simulink model "ray_motor"  (Simulink 7.7)
settings: Solver=FixedStepDiscrete  SolverMode=SingleTasking  StartTime=0.0  StopTime=inf  FixedStep=0.001  RelTol=1e-3
libraries: dsPICdrivers x9, simulink x1
settings Model: Creator=Ray  LastModifiedBy=l45chen
settings OptimizationCC: OptimizeModelRefInitCode=on  LifeSpan=Inf
settings HardwareCC: ProdBitPerInt=16  ProdBitPerPointer=16  ProdEndianess=LittleEndian  ProdWordSize=16  ProdHWDeviceType=16-bit Generic
settings RTWCC: SystemTargetFile=dspic.tlc  MakeCommand=make_CreateMPLAB  TemplateMakefile=dspic_pic30_gcc.tmf  PostCodeGenCommand=dsPIC_Compile()  Description=Embedded Target for Microchip dsPIC (real-time)  ProcessScript=dspic_make_rtw_hook
settings CodeAppCC: IgnoreCustomStorageClasses=off
settings STFCustomTargetCC: FunctionExecutionProfile=off  IncludeMdlTerminateFcn=off  CombineOutputUpdateFcns=on  ERTCustomFileBanners=on  SupportNonInlinedSFcns=off  SystemTargetFile=dspic.tlc
settings ERTTargetCC: FunctionExecutionProfile=off  MultiwordLength=2048  ParMdlRefBuildCompliant=off  CompOptLevelCompliant=off  IncludeMdlTerminateFcn=off  ERTFirstTimeCompliant=off  SupportContinuousTime=on  ModelStepFunctionPrototypeControlCompliant=off  CPPClassGenCompliant=off  ExtModeMexFile=ext_serial_win32_comm  InlinedParameterPlacement=NonHierarchical  ERTSrcFileBannerTemplate=dsPIC_code_template.cgt  ERTHdrFileBannerTemplate=dsPIC_code_template.cgt  ERTDataSrcFileTemplate=dsPIC_code_template.cgt  ERTDataHdrFileTemplate=dsPIC_code_template.cgt  ERTCustomFileTemplate=dsPIC_main.tlc  ConvertIfToSwitch=off
settings CustomProperty: DataType=string  Value=C:\PROGRA~1\MATLAB\R2011a\bin\win64\gmake

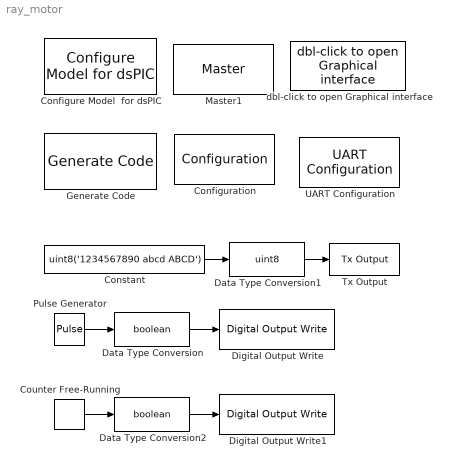
== system ray_motor ==
  Configuration : dsPICdrivers/Configuration  SystemSampleTime=-1  double64=off
  Configure Model  for dsPIC : dsPICdrivers/Simulink Configuration/Configure Model  for dsPIC
  Constant : Constant  Value=uint8('1234567890 abcd ABCD')  OutDataTypeStr=uint8
  Counter Free-Running : simulink/Sources/Counter Free-Running  SystemSampleTime=-1  NumBits=1  tsamp=0.5
  Data Type Conversion : DataTypeConversion  OutDataTypeStr=boolean
  Data Type Conversion1 : DataTypeConversion  OutDataTypeStr=uint8
  Data Type Conversion2 : DataTypeConversion  OutDataTypeStr=boolean
  Digital Output Write : dsPICdrivers/Digital I//O/Digital Output Write  Tag=dsPIC_Digital_Output  Priority=5  PORT=B  Pin=[14]  Simultaneous=off  OrderingInOutPopup=None
  Digital Output Write1 : dsPICdrivers/Digital I//O/Digital Output Write  Tag=dsPIC_Digital_Output  Priority=5  PORT=B  Pin=[15]  Simultaneous=off  OrderingInOutPopup=None
  Generate Code : dsPICdrivers/Simulink Configuration/Generate Code
  Master1 : dsPICdrivers/Master  Tag=dsPIC_MASTER  Priority=1  TimeStepType=Timer1  picType=33fj32MC204  fcy=40000000  Quartz_33f=8e6  PLLActive_33f=on  fcyDesired_33f=40e6  tmr1="[1  39999  0]"  tmr1Info="Time Step : 0.001  ;   Error : 0%  PR1=39999"  tmr2345="[0  0]"  tmr2345cfg=[-1 -1]  IOautoConf=on  typePort="[ 0   0   0   0   0   0   0   0   0   0   0   0   0   0   0   0   0   0   0   0   0   0   0   0   0   0   0   0   0   0  10  10   0   0   0   0   0   0   0   0   0   0   0   0   0   0   0   0   0   0   0   0   0   0   0   0   0   0   0   0   0   0   0   0   0   0   0   0   0   0   0   0   0   0   0   0   0   0   0   0   0   0   0   0   0   0   0   0   0   0   0   0   0   0   0   0   0   0   0   0   0   0   0   0   0   0   0   0   0   0   0   0 ]"  TRIS="[ 65535  16383  65535  65535  65535  65535  65535 ]"  ADPCFG=0  MasterBusyPort=None  MasterOverloadPort=None  FOSC=Quartz (XT - HS)  ClockSwitchMonitor=Both disabled  TempProtection_33f=TEMP_ON  FPBOR=<empty>  PWRT=disable  MCLR=<empty>  ICD=ICS_PGD1  JTAGEN=JTAGEN_OFF  PowerSave=off  OverrideFcy=off  NewFcy=1e6  PR2345="[65535  65535]"
  Pulse Generator : DiscretePulseGenerator  PulseType=Time based  Period=1  PulseWidth=50
  Tx Output : dsPICdrivers/Serial PORT/Tx Output  Tag=dsPIC_TX  Priority=5  UART=1  OrderingInOutPopup=None
  UART Configuration : dsPICdrivers/Serial PORT/UART Configuration  Tag=dsPIC_config_UART  Priority=2  UART=1  proposed_BAUD=38400  BAUD=38400  ALT_TX_RX=on  InterruptTxWhen=When Transmit Buffer is empty  TXInterruptPri=1  TxBufferSize=32  TXEN=on  InterruptRxWhen=When Receive Buffer is full (contain 4 characters)  RXInterruptPri=2  RxBufferSize=32  DoNotImplementRxInterrupt=off  DoNotImplementTxInterrupt=off  UxBRG=64  Info="UxBRG = 64   ||  Real Baud : 38462   ||  % error : 0.16026  ||  max 3.8462 Bytes / Step"  RealBaud=0  ERROR=0.16026  BYTES_STEP=3.8462
  dbl-click to open Graphical interface : dsPICdrivers/Serial PORT/dbl-click to open Graphical interface  Nothing=0
  wires:
  Constant/1 -> Data Type Conversion1/1
  Pulse Generator/1 -> Data Type Conversion/1
  Data Type Conversion/1 -> Digital Output Write/1
  Data Type Conversion1/1 -> Tx Output/1
  Counter Free-Running/1 -> Data Type Conversion2/1
  Data Type Conversion2/1 -> Digital Output Write1/1
